simulink library "Lib_Piccolo"  (R2018b)
settings: Solver=VariableStepAuto  StartTime=0.0  StopTime=10.0  RelTol=1e-3
values from neighbouring files (symbols this model uses):
  AccelErrInt2Brakes = 0.15    [SimulationControlConfig16P.m]    (also in SimulationControlConfig16P_LEGACY.m; SimulationControlConfigTAILLESS.m = 0.2; SimulationControlConfigUTAIL.m = 0.2)
  AileronMax = 25    [SimulationControlConfig16P.m]    (also in SimulationControlConfig16P_LEGACY.m; SimulationControlConfigTAILLESS.m; SimulationControlConfigUTAIL.m)
  AileronPower = 0.00268    [SimulationControlConfig16P.m]    (also in SimulationControlConfig16P_LEGACY.m; SimulationControlConfigTAILLESS.m; SimulationControlConfigUTAIL.m)
  AileronSurfaceMax = 45    [SimulationControlConfig16P.m]    (also in SimulationControlConfig16P_LEGACY.m)
  AileronTrim = 0    [SimulationControlConfig16P.m]    (also in SimulationControlConfig16P_LEGACY.m; SimulationControlConfigTAILLESS.m; SimulationControlConfigUTAIL.m)
  Alt = 1000 + TerrainHeight    [SimulationStateConfig.m]
  AltCruise_m = testPlans(testIndx).terrainElevation * 0.3048 + 200    [SimulationControlConfig16P.m]    (also in SimulationControlConfigTAILLESS.m = 1083; SimulationControlConfigUTAIL.m = testPlans(testIndx).terrainElevation * 0.3048 + 152)
  AltitudeRate2PitchCmdIntegratorInit = 0.1    [SimulationControlPre.m]
  AltMax = 10000    [SimulationControlConfig16P.m]    (also in SimulationControlConfig16P_LEGACY.m; SimulationControlConfigTAILLESS.m; SimulationControlConfigUTAIL.m)
  AltMaxAccel = 1.25    [SimulationControlConfig16P.m]    (also in SimulationControlConfig16P_LEGACY.m = 0.9; SimulationControlConfigTAILLESS.m = 1.7; SimulationControlConfigUTAIL.m = 2)
  AltMin = 0    [SimulationControlConfig16P.m]    (also in SimulationControlConfig16P_LEGACY.m; SimulationControlConfigTAILLESS.m; SimulationControlConfigUTAIL.m)
  AltRateCmd2Pitch = 0.50    (= 0.5)    [SimulationControlConfig16P.m]    (also in SimulationControlConfig16P_LEGACY.m = 0.6; SimulationControlConfigTAILLESS.m = 0.2; SimulationControlConfigUTAIL.m = 0.3)
  AltRateError2Pitch = 0.40    (= 0.4)    [SimulationControlConfig16P.m]    (also in SimulationControlConfig16P_LEGACY.m; SimulationControlConfigTAILLESS.m = 0.55; SimulationControlConfigUTAIL.m = 0.55)
  AltRateErrorInt2Pitch = 0.50    (= 0.5)    [SimulationControlConfig16P.m]    (also in SimulationControlConfig16P_LEGACY.m = 0.45; SimulationControlConfigTAILLESS.m; SimulationControlConfigUTAIL.m = 0.75)
  AltRateLpfCutOff = 3    [SimulationControlConfig16P.m]    (also in SimulationControlConfig16P_LEGACY.m; SimulationControlConfigTAILLESS.m = 2; SimulationControlConfigUTAIL.m = 2)
  AutoNosegear2Rudder = 26    [SimulationControlConfig16P.m]    (also in SimulationControlConfig16P_LEGACY.m; SimulationControlConfigTAILLESS.m = 25.2; SimulationControlConfigUTAIL.m = 14)
  b = 5.54    [SimulationControlConfig16P.m]    (also in SimulationControlConfig16P_LEGACY.m; SimulationControlConfigTAILLESS.m = 2.37; SimulationControlConfigUTAIL.m = 2.37)
  Bank2AileronIntegratorInit = 0    [SimulationControlPre.m]
  BankMax_User = BankMax_User/180*pi    (= 0.523598775598)    [SimulationControlConfig16P.m]    (also in SimulationControlConfig16P_LEGACY.m; SimulationControlConfigTAILLESS.m = 0.610865238198; SimulationControlConfigUTAIL.m = 0.628318530718)
  baseLegFlaps = 20    [SimulationControlConfig16P.m]    (also in SimulationControlConfig16P_LEGACY.m = 0; SimulationControlConfigTAILLESS.m = 15; SimulationControlConfigUTAIL.m = 10)
  C = GeneticOpt.C    [SimulationCostFunction.m]
  c = Sw/b    (= 0.841696750903)    [SimulationControlConfig16P.m]    (also in SimulationControlConfig16P_LEGACY.m; SimulationControlConfigTAILLESS.m = 0.354008438819; SimulationControlConfigUTAIL.m = 0.354008438819)
  cell2WheelFactorMG = 5.98    [SimulationSensorConfig16P_LEGACY.m]
  cell2WheelFactorNG = 1    [SimulationSensorConfig16P_LEGACY.m]
  cellSatMaxMG = 15000    [SimulationSensorConfig16P.m]    (also in SimulationSensorConfig16P_LEGACY.m; SimulationSensorConfigTAILLESS7P.m; SimulationSensorConfigUTAIL7P.m)
  cellSatMaxNG = 1000    [SimulationSensorConfig16P.m]    (also in SimulationSensorConfig16P_LEGACY.m; SimulationSensorConfigTAILLESS7P.m; SimulationSensorConfigUTAIL7P.m)
  cellSatMinMG = -15000    [SimulationSensorConfig16P.m]    (also in SimulationSensorConfig16P_LEGACY.m; SimulationSensorConfigTAILLESS7P.m; SimulationSensorConfigUTAIL7P.m)
  cellSatMinNG = -1000    [SimulationSensorConfig16P.m]    (also in SimulationSensorConfig16P_LEGACY.m; SimulationSensorConfigTAILLESS7P.m; SimulationSensorConfigUTAIL7P.m)
  CL_Limit = CL_Max    (= 0.54)    [SimulationControlConfig16P.m]    (also in SimulationControlConfig16P_LEGACY.m; SimulationControlConfigTAILLESS.m; SimulationControlConfigUTAIL.m = 0.53)
  CL_Max = 0.54    [SimulationControlConfig16P.m]    (also in SimulationControlConfig16P_LEGACY.m; SimulationControlConfigTAILLESS.m; SimulationControlConfigUTAIL.m = 0.53)
  CL_Max_Nom = 0.465    [SimulationControlConfig16P.m]    (also in SimulationControlConfig16P_LEGACY.m; SimulationControlConfigTAILLESS.m = 0.39; SimulationControlConfigUTAIL.m)
  CL_Min = 0    [SimulationControlConfig16P.m]    (also in SimulationControlConfig16P_LEGACY.m; SimulationControlConfigTAILLESS.m; SimulationControlConfigUTAIL.m)
  ClimbMaxFraction = 0.35    [SimulationControlConfig16P.m]    (also in SimulationControlConfig16P_LEGACY.m = 0.24; SimulationControlConfigTAILLESS.m = 0.19; SimulationControlConfigUTAIL.m = 0.21)
  ClimboutMaxBank = 7.0    (= 7)    [SimulationControlConfig16P.m]    (also in SimulationControlConfig16P_LEGACY.m; SimulationControlConfigTAILLESS.m = 5; SimulationControlConfigUTAIL.m)
  ClimboutTimer = 7.0    (= 7)    [SimulationControlConfig16P.m]    (also in SimulationControlConfig16P_LEGACY.m; SimulationControlConfigTAILLESS.m; SimulationControlConfigUTAIL.m)
  dCl_per_dFlap = 0.005581818    [SimulationControlConfig16P.m]    (also in SimulationControlConfig16P_LEGACY.m = 0; SimulationControlConfigTAILLESS.m = 0; SimulationControlConfigUTAIL.m = 0)
  DecelerationCmd = 3.1    [SimulationControlConfig16P.m]    (also in SimulationControlConfig16P_LEGACY.m; SimulationControlConfigTAILLESS.m = 0.1; SimulationControlConfigUTAIL.m = 0.1)
  DeRotateLogicEndTimer = abs((NoseDownLimit_Deg-1)/DeRotateRamp_Dps)    [SimulationControlConfig16P.m]    (also in SimulationControlConfig16P_LEGACY.m; SimulationControlConfigTAILLESS.m; SimulationControlConfigUTAIL.m)
  DeRotateLogicHoldNoseUpTimer = 0.1    [SimulationControlConfig16P.m]    (also in SimulationControlConfig16P_LEGACY.m; SimulationControlConfigTAILLESS.m; SimulationControlConfigUTAIL.m)
  DeRotateLogicTimerTimeout = 2    [SimulationControlConfig16P.m]    (also in SimulationControlConfig16P_LEGACY.m; SimulationControlConfigTAILLESS.m; SimulationControlConfigUTAIL.m)
  DeRotateLowerCmdSaturation = 0    [SimulationControlConfig16P.m]    (also in SimulationControlConfig16P_LEGACY.m; SimulationControlConfigTAILLESS.m; SimulationControlConfigUTAIL.m)
  DeRotateRamp_Dps = 3    [SimulationControlConfig16P.m]    (also in SimulationControlConfig16P_LEGACY.m; SimulationControlConfigTAILLESS.m = 8; SimulationControlConfigUTAIL.m = 8)
  DeRotateUpperCmdSaturation = 7    [SimulationControlConfig16P.m]    (also in SimulationControlConfig16P_LEGACY.m; SimulationControlConfigTAILLESS.m; SimulationControlConfigUTAIL.m)
  DescentMaxFraction = 0.22    [SimulationControlConfig16P.m]    (also in SimulationControlConfig16P_LEGACY.m = 0.2; SimulationControlConfigTAILLESS.m = 0.17; SimulationControlConfigUTAIL.m = 0.17)
  DesktopSimTerrainOffset_m = 0.406    [SimulationAircraftConfig.m]
  downwindFlaps = 0    [SimulationControlConfig16P.m]    (also in SimulationControlConfig16P_LEGACY.m; SimulationControlConfigTAILLESS.m; SimulationControlConfigUTAIL.m)
  DP_init = 0.5*1.225*V_init^2    [SimulationControlConfig16P.m]    (also in SimulationControlConfig16P_LEGACY.m; SimulationControlConfigTAILLESS.m; SimulationControlConfigUTAIL.m)
  dscNoiseMG = 1    [SimulationSensorConfig16P_LEGACY.m]
  dscNoiseNG = 0.25    [SimulationSensorConfig16P_LEGACY.m]
  DSCnumBits = 24    [SimulationSensorConfig16P.m]    (also in SimulationSensorConfig16P_LEGACY.m; SimulationSensorConfigTAILLESS7P.m; SimulationSensorConfigUTAIL7P.m)
  DSCRangeMaxMG = 15000    [SimulationSensorConfig16P.m]    (also in SimulationSensorConfig16P_LEGACY.m; SimulationSensorConfigTAILLESS7P.m; SimulationSensorConfigUTAIL7P.m)
  DSCRangeMaxNG = 1000    [SimulationSensorConfig16P.m]    (also in SimulationSensorConfig16P_LEGACY.m; SimulationSensorConfigTAILLESS7P.m; SimulationSensorConfigUTAIL7P.m)
  DSCRangeMinMG = -15000    [SimulationSensorConfig16P.m]    (also in SimulationSensorConfig16P_LEGACY.m; SimulationSensorConfigTAILLESS7P.m; SimulationSensorConfigUTAIL7P.m)
  DSCRangeMinNG = -1000    [SimulationSensorConfig16P.m]    (also in SimulationSensorConfig16P_LEGACY.m; SimulationSensorConfigTAILLESS7P.m; SimulationSensorConfigUTAIL7P.m)
  dt = DLLSim.dt    [SimulationTimeStep.m]    (also in SimulationTrim.m = 0.02)
  EarlyTouchdownThreshold = 3.0    (= 3)    [SimulationControlConfig16P.m]    (also in SimulationControlConfig16P_LEGACY.m; SimulationControlConfigTAILLESS.m = 2.2; SimulationControlConfigUTAIL.m = 2.5)
  ElevatorDeflectionRate = 15    [SimulationControlConfig16P.m]    (also in SimulationControlConfig16P_LEGACY.m = 12; SimulationControlConfigTAILLESS.m = 10; SimulationControlConfigUTAIL.m = 12)
  ElevatorMax = 25    [SimulationControlConfig16P.m]    (also in SimulationControlConfig16P_LEGACY.m; SimulationControlConfigTAILLESS.m; SimulationControlConfigUTAIL.m)
  ElevatorPower = -0.002209    [SimulationControlConfig16P.m]    (also in SimulationControlConfig16P_LEGACY.m; SimulationControlConfigTAILLESS.m = -0.002956; SimulationControlConfigUTAIL.m = -0.00205983)
  ElevatorTrim = -3.5    [SimulationControlConfig16P.m]    (also in SimulationControlConfig16P_LEGACY.m; SimulationControlConfigTAILLESS.m = -6; SimulationControlConfigUTAIL.m = -8)
  elevonBias = 0    [SimulationControlConfig16P.m]    (also in SimulationControlConfig16P_LEGACY.m; SimulationControlConfigTAILLESS.m; SimulationControlConfigUTAIL.m)
  Enable_TAS_Protection = 0    [SimulationControlConfig16P.m]    (also in SimulationControlConfig16P_LEGACY.m; SimulationControlConfigTAILLESS.m; SimulationControlConfigUTAIL.m)
  EnableCrossTrackAbort = 1    [SimulationControlConfig16P.m]    (also in SimulationControlConfigTAILLESS.m; SimulationControlConfigUTAIL.m)
  EnergyBandwidth = 0.02    [SimulationControlConfig16P.m]    (also in SimulationControlConfig16P_LEGACY.m; SimulationControlConfigTAILLESS.m = 0.06; SimulationControlConfigUTAIL.m = 0.06)
  EngineLhFuelCut = 0    [SimulationAircraftConfig.m]
  EngineRhFuelCut = 0    [SimulationAircraftConfig.m]
  FastThrottleRate = 0.075    [SimulationControlConfig16P.m]    (also in SimulationControlConfig16P_LEGACY.m = 0.05; SimulationControlConfigTAILLESS.m = 0.1; SimulationControlConfigUTAIL.m = 0.1)
  FilterWarmUpTime = 2    [SimulationSensorConfig16P.m]    (also in SimulationSensorConfig16P_LEGACY.m; SimulationSensorConfigTAILLESS7P.m; SimulationSensorConfigUTAIL7P.m)
  finalApproachFlaps = 20    [SimulationControlConfig16P.m]    (also in SimulationControlConfig16P_LEGACY.m = 0; SimulationControlConfigTAILLESS.m = 22; SimulationControlConfigUTAIL.m = 10)
  FinalDescentSlope_Deg = testPlans(testIndx).descentSlope    [SimulationControlConfig16P.m]    (also in SimulationControlConfig16P_LEGACY.m; SimulationControlConfigTAILLESS.m; SimulationControlConfigUTAIL.m)
  flapMax = 0    [SimulationControlConfig16P.m]    (also in SimulationControlConfig16P_LEGACY.m; SimulationControlConfigTAILLESS.m; SimulationControlConfigUTAIL.m)
  flapRate = 7.5    [SimulationControlConfig16P.m]    (also in SimulationControlConfig16P_LEGACY.m; SimulationControlConfigTAILLESS.m = 6.6; SimulationControlConfigUTAIL.m)
  FlareHeight = 5    [SimulationControlConfig16P.m]    (also in SimulationControlConfig16P_LEGACY.m = 4.8; SimulationControlConfigTAILLESS.m = 2.5; SimulationControlConfigUTAIL.m = 2)
  FlareVerticalRate_mps = -0.4    [SimulationControlConfig16P.m]    (also in SimulationControlConfig16P_LEGACY.m = -0.5; SimulationControlConfigTAILLESS.m = -0.15; SimulationControlConfigUTAIL.m = -0.15)
  Fp_Aileron = 0.55*2*pi*RollRateLpfCutoff*dt    [SimulationControlConfig16P.m]    (also in SimulationControlConfig16P_LEGACY.m; SimulationControlConfigTAILLESS.m; SimulationControlConfigUTAIL.m)
  Fp_Alt = 0.55*AltBandwidth    (= 0.099)    [SimulationControlConfig16P.m]    (also in SimulationControlConfig16P_LEGACY.m; SimulationControlConfigTAILLESS.m = 0.587477826221; SimulationControlConfigUTAIL.m = 0.69115038379)
  Fp_AltRate = 0.55*2*pi*AltRateLpfCutOff*dt    [SimulationControlConfig16P.m]    (also in SimulationControlConfig16P_LEGACY.m; SimulationControlConfigTAILLESS.m; SimulationControlConfigUTAIL.m)
  Fp_Elevator = 0.55*2*pi*PitchRateLpfCutoff*dt    [SimulationControlConfig16P.m]    (also in SimulationControlConfig16P_LEGACY.m; SimulationControlConfigTAILLESS.m; SimulationControlConfigUTAIL.m)
  Fp_Energy = 0.55*2*pi*EnergyBandwidth    (= 0.069115038379)    [SimulationControlConfig16P.m]    (also in SimulationControlConfig16P_LEGACY.m; SimulationControlConfigTAILLESS.m = 0.207345115137; SimulationControlConfigUTAIL.m = 0.207345115137)
  Fp_Energy2 = 0.55*2*pi*EnergyBandwidth*dt    [SimulationControlConfig16P.m]    (also in SimulationControlConfig16P_LEGACY.m; SimulationControlConfigTAILLESS.m; SimulationControlConfigUTAIL.m)
  Fp_Pitch = 0.55*2*pi*PitchBandwidth    (= 2.76460153516)    [SimulationControlConfig16P.m]    (also in SimulationControlConfig16P_LEGACY.m = 3.11017672705; SimulationControlConfigTAILLESS.m = 3.80132711084; SimulationControlConfigUTAIL.m = 2.41902634326)
  Fp_Pitch_2 = 0.55*2*pi*PitchBandwidth*dt    [SimulationControlConfig16P.m]    (also in SimulationControlConfig16P_LEGACY.m; SimulationControlConfigTAILLESS.m; SimulationControlConfigUTAIL.m)
  Fp_Roll = RollBandwidth^2    (= 1)    [SimulationControlConfig16P.m]    (also in SimulationControlConfig16P_LEGACY.m = 1.44; SimulationControlConfigTAILLESS.m; SimulationControlConfigUTAIL.m)
  Fp_Rudder = 0.55*2*pi*YawRateLpfCutoff*dt    [SimulationControlConfig16P.m]    (also in SimulationControlConfig16P_LEGACY.m; SimulationControlConfigTAILLESS.m; SimulationControlConfigUTAIL.m)
  Fp_TAS = 0.55*2*pi*TASBandwidth    (= 0.103672557568)    [SimulationControlConfig16P.m]    (also in SimulationControlConfig16P_LEGACY.m; SimulationControlConfigTAILLESS.m = 0.172787595947; SimulationControlConfigUTAIL.m = 0.172787595947)
  Fp_TAS_Filter = 2*pi*TasLpfCutoff*dt    [SimulationControlConfig16P.m]    (also in SimulationControlConfig16P_LEGACY.m; SimulationControlConfigTAILLESS.m; SimulationControlConfigUTAIL.m)
  Fp_Turn = 0.55*2*pi*TurnErrLPFcutoff    (= 0.0345575191895)    [SimulationControlConfig16P.m]    (also in SimulationControlConfig16P_LEGACY.m; SimulationControlConfigTAILLESS.m = 0.172787595947; SimulationControlConfigUTAIL.m = 0.172787595947)
  Fp_TurnDerr = 0.55*2*pi*TurnDerivativeLPFcutoff    (= 0.0345575191895)    [SimulationControlConfig16P.m]    (also in SimulationControlConfig16P_LEGACY.m; SimulationControlConfigTAILLESS.m = 0.172787595947; SimulationControlConfigUTAIL.m = 0.172787595947)
  FTV = 3    [SimulationAircraftConfig.m]
  ftvStaticPositionError = 1/1.18    (= 0.847457627119)    [SimulationSensorConfig16P.m]    (also in SimulationSensorConfig16P_LEGACY.m; SimulationSensorConfigTAILLESS7P.m = 1; SimulationSensorConfigUTAIL7P.m = 1)
  g = 9.81    [SimulationStateConfig.m]
  GustSpd_Kts = testPlans(testIndx).gustSpd    [SimulationStateConfig.m]
  GustTriggerVal = testPlans(testIndx).gustTriggerVal    [SimulationStateConfig.m]
  HeadingErr2TurnRate = 0.5    [SimulationControlConfig16P.m]    (also in SimulationControlConfig16P_LEGACY.m; SimulationControlConfigTAILLESS.m; SimulationControlConfigUTAIL.m)
  HeadingErrDer2TurnRate = 0.3    [SimulationControlConfig16P.m]    (also in SimulationControlConfig16P_LEGACY.m; SimulationControlConfigTAILLESS.m; SimulationControlConfigUTAIL.m)
  IASbounce = IASstall*0.8    [SimulationControlPre.m]
  IAScruiseCMD = sqrt(2*m*9.81/(1.225*Sw*CL_cruise))    [SimulationControlConfig16P.m]    (also in SimulationControlConfig16P_LEGACY.m; SimulationControlConfigTAILLESS.m; SimulationControlConfigUTAIL.m)
  IASfinalCMD = 1.12 * IASmin    [SimulationControlConfig16P.m]    (also in SimulationControlConfig16P_LEGACY.m = 1.10 * IASmin; SimulationControlConfigTAILLESS.m = 1.10 * IASmin; SimulationControlConfigUTAIL.m = 1.15 * IASmin)
  IASflareCMD = IASstall    [SimulationControlConfig16P.m]    (also in SimulationControlConfig16P_LEGACY.m; SimulationControlConfigTAILLESS.m; SimulationControlConfigUTAIL.m)
  IASmax = 64    [SimulationControlConfig16P.m]    (also in SimulationControlConfig16P_LEGACY.m = 46; SimulationControlConfigTAILLESS.m = 38.58; SimulationControlConfigUTAIL.m = 35)
  IASmin = sqrt(2*m*9.81/(1.225*Sw*0.9*CL_Max_Nom))    [SimulationControlConfig16P.m]    (also in SimulationControlConfig16P_LEGACY.m; SimulationControlConfigTAILLESS.m; SimulationControlConfigUTAIL.m)
  IASshortCMD = IASstall    [SimulationControlConfig16P.m]    (also in SimulationControlConfig16P_LEGACY.m; SimulationControlConfigTAILLESS.m; SimulationControlConfigUTAIL.m)
  IASstall = sqrt(2*m*9.81/(1.225*Sw*CL_Max))    [SimulationControlConfig16P.m]    (also in SimulationControlConfig16P_LEGACY.m; SimulationControlConfigTAILLESS.m; SimulationControlConfigUTAIL.m)
  inFlight = 1    [SimulationControlConfig16P.m]    (also in SimulationControlConfigTAILLESS.m; SimulationControlConfigUTAIL.m)
  JetCatOffset = 5    [SimulationControlConfig16P.m]    (also in SimulationControlConfig16P_LEGACY.m)
  LaunchRollingElevator = -1.5    [SimulationControlConfig16P.m]    (also in SimulationControlConfig16P_LEGACY.m; SimulationControlConfigTAILLESS.m = 1; SimulationControlConfigUTAIL.m = 1)
  ldg_NosegearMax = 10    [SimulationControlConfig16P.m]    (also in SimulationControlConfig16P_LEGACY.m; SimulationControlConfigTAILLESS.m; SimulationControlConfigUTAIL.m)
  ldg_TrackVyErrInt2Nosegear = 0.1250    (= 0.125)    [SimulationControlConfig16P.m]    (also in SimulationControlConfig16P_LEGACY.m; SimulationControlConfigTAILLESS.m = 0.00714285714286; SimulationControlConfigUTAIL.m = 0.00714285714286)
  ldg_TrackVyErrPro2Nosegear = 0.35    [SimulationControlConfig16P.m]    (also in SimulationControlConfig16P_LEGACY.m; SimulationControlConfigTAILLESS.m = 0.0546666666667; SimulationControlConfigUTAIL.m = 0.0546666666667)
  ldg_TrackY2Vy = 0.07    [SimulationControlConfig16P.m]    (also in SimulationControlConfig16P_LEGACY.m; SimulationControlConfigTAILLESS.m = 0.17; SimulationControlConfigUTAIL.m = 0.17)
  ldg_Vy2NosegearScalingPower = 1.075    [SimulationControlConfig16P.m]    (also in SimulationControlConfig16P_LEGACY.m; SimulationControlConfigTAILLESS.m = 0.6; SimulationControlConfigUTAIL.m = 0.5)
  ldg_Y2VyScalingPower = 0.175    [SimulationControlConfig16P.m]    (also in SimulationControlConfig16P_LEGACY.m; SimulationControlConfigTAILLESS.m = 0; SimulationControlConfigUTAIL.m = 0)
  ldg_YawRate2Nosegear = 0.175    [SimulationControlConfig16P.m]    (also in SimulationControlConfig16P_LEGACY.m; SimulationControlConfigTAILLESS.m = 0.065; SimulationControlConfigUTAIL.m = 0.065)
  LiftSlope = 0.064285    [SimulationControlConfig16P.m]    (also in SimulationControlConfig16P_LEGACY.m; SimulationControlConfigTAILLESS.m = 0.058631; SimulationControlConfigUTAIL.m)
  LPFaileronInit = 0    [SimulationControlPre.m]
  LPFclestInit = 0    [SimulationControlPre.m]
  LPFenergyFFInit = 0    [SimulationControlPre.m]
  LPFtasInit = V_init + 2    [SimulationControlPre.m]
  LPFthrottleInit = ThrottleTrim    [SimulationControlPre.m]
  LPFturnErrInit = 0    [SimulationControlPre.m]
  ... (+115 more)
undefined symbols (not defined in the file or in its folder): abortFlag, alphaHPF, apmDelay, BRWNOUT, CRAWOR, CRAWUR, DiscIntNeverNeededParam, DLLSim, DLLSimStep, ECOMOR, ECOMUR, Fp_Tas, GustTrigger_HeightAgl_m, IPSTAT, LCINTEG, Ldg_Persist_Time, LOWER_FLAGS, MSG_ENABLE, NoiseStd, OLDVAL, OVERRIDE_ENABLE, OVERRIDE_VALUE, REBOOT, reversionEnable, revIASMax, revIASMin, revPitchMax, revPitchMin, revPitchRateMax, revRollMax, revRollRateMax, SAMPLE, SCALON, SensorModel, sigbuilder_block, Sim_Vx, Sim_Vy, Sim_Vz, Sim_Xpos, Sim_Ypos, Sim_Zpos, SYSOR, SYSUR, TARE, TEMPOR, TEMPUR, testIndx, testPlan, testPlans, Trim_piccoloInCmd, Trim_REFSI_FD_IN_nmodeCgShifterCmd_Ft, Trim_REFSI_FD_IN_nmodeFlapLhIBCmd_Deg, Trim_REFSI_FD_IN_nmodeFlapLhOBCmd_Deg, Trim_REFSI_FD_IN_nmodeFlapRhIBCmd_Deg, Trim_REFSI_FD_IN_nmodeFlapRhOBCmd_Deg, Trim_REFSI_FD_IN_nmodeSlatLhCmd_Deg, Trim_REFSI_FD_IN_nmodeSlatRhCmd_Deg, Trim_REFSI_FD_IN_nmodeSplrLhInbdCmd_Deg, Trim_REFSI_FD_IN_nmodeSplrLhOutbdCmd_Deg ... (+5)
libraries: simulink x866, aerolibconvert2 x60, $bdroot x52, aerolibatmos2 x5, dspswit3 x5, simulink_extras x4, dsparch4 x2, Lib_Piccolo_Alt x2, eeGeneralControl x1, dspindex x1
(part 12 of 44)

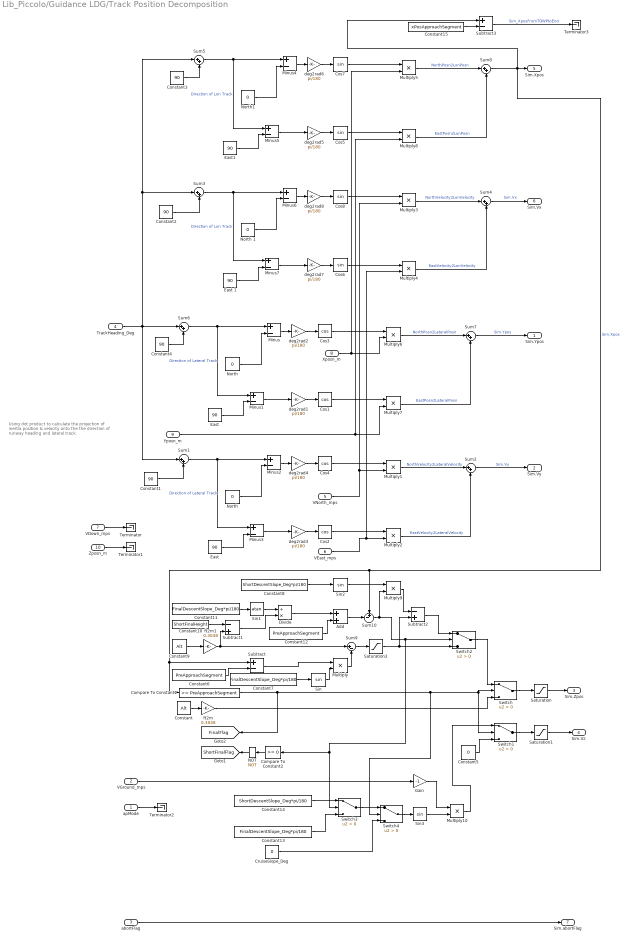
== system Lib_Piccolo/Guidance LDG/Track Position Decomposition ==
  note: Using dot product to calculate the projection of inertia position & velocity onto the
      | the direction of runway heading and lateral track
  apMode : Inport
  VGround_mps : Inport  Port=2
  abortFlag : Inport  Port=3
  TrackHeading_Deg : Inport  Port=4
  VNorth_mps : Inport  Port=5
  VEast_mps : Inport  Port=6
  VDown_mps : Inport  Port=7
  "Xposn_m " : Inport  Port=8
  Yposn_m : Inport  Port=9
  Zposn_m : Inport  Port=10
  Add : Sum
  Compare To Constant1 : simulink/Logic and Bit Operations/Compare To Constant  relop=>=  const=PreApproachSegment  OutDataTypeStr=uint8
  Compare To Constant2 : simulink/Logic and Bit Operations/Compare To Constant  relop=>=  const=0  OutDataTypeStr=uint8
  Constant : Constant  Value=Alt
  Constant{1..4} (4 alike) : Constant  Value=90
  Constant10 : Constant  Value=ShortFinalHeight
  Constant11 : Constant  Value=FinalDescentSlope_Deg*pi/180
  Constant12 : Constant  Value=PreApproachSegment
  Constant13 : Constant  Value=FinalDescentSlope_Deg*pi/180
  Constant14 : Constant  Value=ShortDescentSlope_Deg*pi/180
  Constant15 : Constant  Value=xPosApproachSegment
  Constant5 : Constant  Value=0
  Constant6 : Constant  Value=PreApproachSegment
  Constant7 : Constant  Value=FinalDescentSlope_Deg*pi/180
  Constant8 : Constant  Value=ShortDescentSlope_Deg*pi/180
  Constant9 : Constant  Value=Alt
  Cos{1..4} (4 alike) : Trigonometry  Operator=cos
  Cos{5..8} (4 alike) : Trigonometry
  CruiseSlope_Deg : Constant  Value=0
  Divide : Product  Inputs=/*
  East : Constant  Value=90
  "East " : Constant  Value=90
  East 1 : Constant  Value=90
  East1 : Constant  Value=90
  Gain : Gain  Gain=-1
  Minus{,1..7} (8 alike) : Sum  Inputs=+-
  Multiply{,1..10} (11 alike) : Product
  NOT : Logic  Operator=NOT  IconShape=distinctive  AllPortsSameDT=off  OutDataTypeStr=boolean
  North : Constant  Value=0
  "North " : Constant  Value=0
  North 1 : Constant  Value=0
  North1 : Constant  Value=0
  Saturation : Saturate  UpperLimit=AltMax  LowerLimit=TerrainHeight*0.3048
  Saturation1 : Saturate  UpperLimit=100  LowerLimit=-100
  Saturation2 : Saturate  UpperLimit=AltMax  LowerLimit=ShortFinalHeight
  Sin : Trigonometry
  Sin1 : Trigonometry  Operator=atan
  Sin2 : Trigonometry
  Sin3 : Trigonometry
  Subtract : Sum  Inputs=+-
  Subtract1 : Sum  Inputs=-+
  Subtract2 : Sum  Inputs=-+
  Subtract3 : Sum  Inputs=+-
  Sum{1..8} (8 alike) : Sum  Inputs=|++
  Sum10 : Sum  Inputs=+-|
  Sum9 : Sum  Inputs=|+-
  Switch{,1..4} (5 alike) : Switch  Criteria=u2 > Threshold
  Terminator{,1..3} (4 alike) : Terminator
  deg2rad{1..8} (8 alike) : Gain  Gain=pi/180
  ft2m : Gain  Gain=0.3048
  ft2m1 : Gain  Gain=0.3048
  Sim.Ypos : Outport
  "Sim.Vy " : Outport  Port=2
  Sim.Zpos : Outport  Port=3
  Sim.Vz : Outport  Port=4
  Sim.Xpos : Outport  Port=5
  Sim.Vx : Outport  Port=6
  Sim.abortFlag : Outport  Port=7
  tag scope: FinalFlag=global, ShortFinalFlag=global
  wires:
  Subtract3/1 -> Terminator3/1  "Sim_XposFromTDWPtoEnd"
  Constant15/1 -> Subtract3/2
  Cos1/1 -> Multiply7/1
  Yposn_m/1 -> Multiply8/2, Multiply7/2
  Multiply7/1 -> Sum7/2  "EastPosn2LateralPosn"
  Multiply6/1 -> Sum7/1  "NorthPosn2LateralPosn"
  Sum6/1 -> Minus/1, Minus1/1  "Direction of Lateral Track"
  Constant4/1 -> Sum6/2
  Cos3/1 -> Multiply6/1
  "Xposn_m "/1 -> Multiply5/2, Multiply6/2
  Sum7/1 -> Sim.Ypos/1  "Sim.Ypos"
  North/1 -> Minus/2
  Minus/1 -> deg2rad2/1
  Minus1/1 -> deg2rad1/1
  East/1 -> Minus1/2
  deg2rad2/1 -> Cos3/1
  deg2rad1/1 -> Cos1/1
  Sum2/1 -> "Sim.Vy "/1  "Sim.Vy"
  VNorth_mps/1 -> Multiply3/2, Multiply1/2
  Constant1/1 -> Sum1/2
  Cos4/1 -> Multiply1/1
  Multiply2/1 -> Sum2/2  "EastVelocity2LateralVelocity"
  Multiply1/1 -> Sum2/1  "NorthVelocity2LateralVelocity"
  VEast_mps/1 -> Multiply4/2, Multiply2/2
  Minus2/1 -> deg2rad4/1
  "North "/1 -> Minus2/2
  Minus3/1 -> deg2rad3/1
  "East "/1 -> Minus3/2
  deg2rad3/1 -> Cos2/1
  Sum1/1 -> Minus2/1, Minus3/1  "Direction of Lateral Track"
  deg2rad4/1 -> Cos4/1
  Cos2/1 -> Multiply2/1
  Constant/1 -> ft2m/1
  Zposn_m/1 -> Terminator1/1
  Minus7/1 -> deg2rad7/1
  Multiply8/1 -> Sum8/2  "EastPosn2LonPosn"
  Cos6/1 -> Multiply4/1
  deg2rad8/1 -> Cos8/1
  deg2rad7/1 -> Cos6/1
  Minus4/1 -> deg2rad6/1
  Minus5/1 -> deg2rad5/1
  Sum3/1 -> Minus6/1, Minus7/1  "Direction of Lon Track"
  TrackHeading_Deg/1 -> Sum6/1, Sum3/1, Sum5/1, Sum1/1
  North 1/1 -> Minus6/2
  Constant3/1 -> Sum5/2
  North1/1 -> Minus4/2
  East1/1 -> Minus5/2
  Constant2/1 -> Sum3/2
  Cos8/1 -> Multiply3/1
  deg2rad5/1 -> Cos5/1
  Sum5/1 -> Minus4/1, Minus5/1  "Direction of Lon Track"
  deg2rad6/1 -> Cos7/1
  Minus6/1 -> deg2rad8/1
  Multiply5/1 -> Sum8/1  "NorthPosn2LonPosn"
  Cos5/1 -> Multiply8/1
  East 1/1 -> Minus7/2
  Multiply3/1 -> Sum4/1  "NorthVelocity2LonVelocity"
  Cos7/1 -> Multiply5/1
  Multiply4/1 -> Sum4/2  "EastVelocity2LonVelocity"
  Sum8/1 -> Sum10/1, Compare To Constant1/1, Subtract/1, Sim.Xpos/1, Subtract3/1  "Sim.Xpos"
  Sum4/1 -> Sim.Vx/1  "Sim.Vx"
  Saturation/1 -> Sim.Zpos/1
  ft2m/1 -> Switch/3
  Constant5/1 -> Switch1/3
  Saturation1/1 -> Sim.Vz/1
  Switch1/1 -> Saturation1/1
  Switch/1 -> Saturation/1
  Constant6/1 -> Subtract/2
  Constant7/1 -> Sin/1
  Subtract/1 -> Multiply/1
  Sin/1 -> Multiply/2
  Constant9/1 -> ft2m1/1
  ft2m1/1 -> Subtract1/2, Sum9/1
  Multiply/1 -> Sum9/2
  Sum9/1 -> Saturation2/1
  Constant10/1 -> Subtract1/1
  Constant11/1 -> Sin1/1
  Sin1/1 -> Divide/1
  Subtract1/1 -> Divide/2
  VDown_mps/1 -> Terminator/1
  Divide/1 -> Add/1
  Constant12/1 -> Add/2
  Add/1 -> Sum10/2
  Saturation2/1 -> Subtract2/2, Switch2/3
  Constant8/1 -> Sin2/1
  Sin2/1 -> Multiply9/1
  Sum10/1 -> Switch3/2, Compare To Constant2/1, Switch2/2, Multiply9/2
  Multiply9/1 -> Subtract2/1
  Subtract2/1 -> Switch2/1
  Switch2/1 -> Switch/1
  Switch3/1 -> Switch4/1
  CruiseSlope_Deg/1 -> Switch4/3
  Switch4/1 -> Sin3/1
  VGround_mps/1 -> Gain/1
  Sin3/1 -> Multiply10/2
  Gain/1 -> Multiply10/1
  Multiply10/1 -> Switch1/1
  Constant14/1 -> Switch3/1
  Constant13/1 -> Switch3/3
  apMode/1 -> Terminator2/1
  Compare To Constant2/1 -> NOT/1
  NOT/1 -> [ShortFinalFlag]
  abortFlag/1 -> Sim.abortFlag/1
  Compare To Constant1/1 -> Switch4/2, Switch/2, Switch1/2, [FinalFlag]

== system Lib_Piccolo/Guidance Takeoff & Flight/Track Position Decomposition ==
  apMode : Inport
  VGround_mps : Inport  Port=2
  abortFlag : Inport  Port=3
  TrackHeading_Deg : Inport  Port=4
  VNorth_mps : Inport  Port=5
  VEast_mps : Inport  Port=6
  VDown_mps : Inport  Port=7
  "Xposn_m " : Inport  Port=8
  Yposn_m : Inport  Port=9
  Zposn_m : Inport  Port=10
  Flight Guidance : Subsystem
  Landing Guidance : Subsystem
  Terminator{,1..8} (9 alike) : Terminator
  Sim.Ypos : Outport
  "Sim.Vy " : Outport  Port=2
  Sim.Zpos : Outport  Port=3
  Sim.Vz : Outport  Port=4
  Sim.Xpos : Outport  Port=5
  Sim.Vx : Outport  Port=6
  Sim.abortFlag : Outport  Port=7
  wires:
  Zposn_m/1 -> Terminator1/1
  VDown_mps/1 -> Terminator/1
  apMode/1 -> Terminator2/1
  abortFlag/1 -> Sim.abortFlag/1
  TrackHeading_Deg/1 -> Landing Guidance/1(TrackHeading_Deg), Flight Guidance/1(TrackHeading_Deg)  "TrackHeading_Deg"
  "Xposn_m "/1 -> Landing Guidance/2(Xposn_m), Flight Guidance/2(Xposn_m)  "Xposn_m"
  Yposn_m/1 -> Landing Guidance/3(Yposn_m), Flight Guidance/3(Yposn_m)  "Yposn_m"
  VNorth_mps/1 -> Landing Guidance/4(VNorth_mps), Flight Guidance/4(VNorth_mps)
  VEast_mps/1 -> Landing Guidance/5(VEast_mps), Flight Guidance/5(VEast_mps)
  VGround_mps/1 -> Landing Guidance/6(VGround_mps), Flight Guidance/6(VGround_mps)  "VGround_mps"
  Flight Guidance/1(Sim.Xpos) -> Sim.Xpos/1
  Flight Guidance/2(Sim.Vx) -> Sim.Vx/1
  Flight Guidance/3(Sim.Ypos) -> Sim.Ypos/1
  Flight Guidance/4(Sim.Vy) -> "Sim.Vy "/1
  Flight Guidance/5(Sim.Zpos) -> Sim.Zpos/1
  Flight Guidance/6(Sim.Vz) -> Sim.Vz/1
  Landing Guidance/1(Sim.Xpos) -> Terminator3/1
  Landing Guidance/2(Sim.Vx) -> Terminator4/1
  Landing Guidance/3(Sim.Ypos) -> Terminator5/1
  Landing Guidance/4(Sim.Vy) -> Terminator6/1
  Landing Guidance/5(Sim.Zpos) -> Terminator7/1
  Landing Guidance/6(Sim.Vz) -> Terminator8/1

== system Lib_Piccolo/Heading Control/LPF Heading ==
  Input : Inport
  Reset : Inport  Port=2
  Add1 : Sum  Inputs=++|
  Compare To Constant2 : simulink/Logic and Bit Operations/Compare To Constant  relop=>  const=0  OutDataTypeStr=uint8
  Constant11 : Constant  Value=TurnErrLPFcutoff
  Switch1 : Switch  Criteria=u2 > Threshold
  Unit Delay1 : UnitDelay  InitialCondition=LPFturnErrInit  SampleTime=-1
  a1 : Gain  Gain=1-Fp_Turn
  b0 : Gain  Gain=Fp_Turn
  Output : Outport
  wires:
  Constant11/1 -> Compare To Constant2/1
  Compare To Constant2/1 -> Switch1/2
  Switch1/1 -> Output/1
  Input/1 -> b0/1, Switch1/3
  Add1/1 -> Switch1/1, Unit Delay1/1
  a1/1 -> Add1/1
  b0/1 -> Add1/2
  Unit Delay1/1 -> a1/1

== system Lib_Piccolo/Heading Control/LPF HeadingDerivative ==
  Input : Inport
  Reset : Inport  Port=2
  Add1 : Sum  Inputs=++|
  Compare To Constant2 : simulink/Logic and Bit Operations/Compare To Constant  relop=>  const=0  OutDataTypeStr=uint8
  Constant11 : Constant  Value=TurnDerivativeLPFcutoff
  Switch1 : Switch  Criteria=u2 > Threshold
  Unit Delay1 : UnitDelay  SampleTime=-1
  a1 : Gain  Gain=1-Fp_TurnDerr
  b0 : Gain  Gain=Fp_TurnDerr
  Output : Outport
  wires:
  Constant11/1 -> Compare To Constant2/1
  Compare To Constant2/1 -> Switch1/2
  Switch1/1 -> Output/1
  Input/1 -> b0/1, Switch1/3
  Add1/1 -> Switch1/1, Unit Delay1/1
  a1/1 -> Add1/1
  b0/1 -> Add1/2
  Unit Delay1/1 -> a1/1

== system Lib_Piccolo/Heading Control/On Ground ==
  GuidanceBankCmd : Inport
  <apMode> : Inport  Port=2
  Compare To Constant1 : simulink/Logic and Bit Operations/Compare To Constant  relop=<=  const=1  OutDataTypeStr=uint8
  Compare To Constant2 : simulink/Logic and Bit Operations/Compare To Constant  relop===  const=11  OutDataTypeStr=uint8
  GroundBankCmd : Constant  Value=0
  OR : Logic  Operator=OR  IconShape=distinctive  AllPortsSameDT=off  OutDataTypeStr=boolean
  Switch : Switch  Criteria=u2 > Threshold
  BankCmd : Outport
  wires:
  Compare To Constant2/1 -> OR/1
  <apMode>/1 -> Compare To Constant1/1, Compare To Constant2/1
  GroundBankCmd/1 -> Switch/1
  GuidanceBankCmd/1 -> Switch/3
  Switch/1 -> BankCmd/1
  OR/1 -> Switch/2
  Compare To Constant1/1 -> OR/2

== system Lib_Piccolo/Heading Control/UnwindHdg ==
  REF.yaw : Inport
  Compare To Constant3 : simulink/Logic and Bit Operations/Compare To Constant  relop=>  const=180  OutDataTypeStr=boolean
  Constant : Constant  Value=360
  Subtract : Sum  Inputs=+-
  Switch : Switch  Criteria=u2 > Threshold
  Out1 : Outport
  wires:
  REF.yaw/1 -> Subtract/1, Compare To Constant3/1, Switch/3
  Compare To Constant3/1 -> Switch/2
  Switch/1 -> Out1/1
  Constant/1 -> Subtract/2
  Subtract/1 -> Switch/1

== system Lib_Piccolo/Heading Control/UnwindHdg1 ==
  REF.yaw : Inport
  Compare To Constant3 : simulink/Logic and Bit Operations/Compare To Constant  relop=>  const=180  OutDataTypeStr=boolean
  Constant : Constant  Value=360
  Subtract : Sum  Inputs=+-
  Switch : Switch  Criteria=u2 > Threshold
  Out1 : Outport
  wires:
  REF.yaw/1 -> Subtract/1, Compare To Constant3/1, Switch/3
  Compare To Constant3/1 -> Switch/2
  Switch/1 -> Out1/1
  Constant/1 -> Subtract/2
  Subtract/1 -> Switch/1

== system Lib_Piccolo/Heading Control/WindCorrectionEstimate ==
  WindSouth : Inport
  WindWest : Inport  Port=2
  Rad2Deg : Gain  Gain=180/pi
  Sqrt : Sqrt  SaturateOnIntegerOverflow=on
  Square : Math  Operator=square  SaturateOnIntegerOverflow=on
  Square1 : Math  Operator=square  SaturateOnIntegerOverflow=on
  Subtract : Sum
  Trigonometric Function2 : Trigonometry  Operator=atan2
  WindMag : Outport
  WindDir : Outport  Port=2
  wires:
  WindSouth/1 -> Square/1, Trigonometric Function2/2
  Square/1 -> Subtract/1
  Square1/1 -> Subtract/2
  Subtract/1 -> Sqrt/1
  Sqrt/1 -> WindMag/1  "Sim.WindMagnitude"
  WindWest/1 -> Square1/1, Trigonometric Function2/1
  Trigonometric Function2/1 -> Rad2Deg/1
  Rad2Deg/1 -> WindDir/1  "Sim.WindDirection"

== system Lib_Piccolo/LDG TAS Cmd/CAS2TAS ==
  In1 : Inport
  Bus Selector2 : BusSelector  OutputSignals=airDensity_kgm
  Constant : Constant  Value=1.225
  Divide : Product  Inputs=*/
  Sqrt : Sqrt  SaturateOnIntegerOverflow=on
  Out1 : Outport
  wires:
  In1/1 -> Bus Selector2/1
  Bus Selector2/1 -> Divide/2  "<airDensity_kgm>"
  Constant/1 -> Divide/1
  Divide/1 -> Sqrt/1
  Sqrt/1 -> Out1/1

== system Lib_Piccolo/LDG TAS Cmd No Offset/CAS2TAS ==
  In1 : Inport
  Bus Selector2 : BusSelector  OutputSignals=airDensity_kgm
  Constant : Constant  Value=1.225
  Divide : Product  Inputs=*/
  Sqrt : Sqrt  SaturateOnIntegerOverflow=on
  Out1 : Outport
  wires:
  In1/1 -> Bus Selector2/1
  Bus Selector2/1 -> Divide/2  "<airDensity_kgm>"
  Constant/1 -> Divide/1
  Divide/1 -> Sqrt/1
  Sqrt/1 -> Out1/1

== system Lib_Piccolo/Piccolo State Machine/Flight State Machine ==
  <apMode> : Inport
  IAS : Inport  Port=2
  GroundSpeed : Inport  Port=3
  AND : Logic  IconShape=distinctive  AllPortsSameDT=off  OutDataTypeStr=boolean
  AND1 : Logic  IconShape=distinctive  AllPortsSameDT=off  OutDataTypeStr=boolean
  Abort Logic : Subsystem
  Compare To Constant : simulink/Logic and Bit Operations/Compare To Constant  relop===  const=0  OutDataTypeStr=boolean
  Compare To Constant1 : simulink/Logic and Bit Operations/Compare To Constant  relop===  const=3.0  OutDataTypeStr=boolean
  Compare To Constant2 : simulink/Logic and Bit Operations/Compare To Constant  relop=>=  const=ClimboutTimer  OutDataTypeStr=boolean
  Compare To Constant3 : simulink/Logic and Bit Operations/Compare To Constant  relop=>=  const=0.75*IASmin  OutDataTypeStr=boolean
  Compare To Constant4 : simulink/Logic and Bit Operations/Compare To Constant  relop=>=  const=RotationSpeed  OutDataTypeStr=boolean
  Constant : Constant  Value=2
  Constant{1,3,5..6} (4 alike) : Constant
  Constant2 : Constant  Value=3
  Constant4 : Constant  Value=4
  Constant9 : Constant  Value=11
  Latch : Subsystem
  Latch1 : Subsystem
  Latch2 : Subsystem
  Switch{,1..3} (4 alike) : Switch  Criteria=u2 > Threshold
  Switch4 : Switch  Criteria=u2 > Threshold  Threshold=0.5
  Timer : Subsystem  mask{period=3}
      mask prompts: period "Period [s]"
  Unit Delay : UnitDelay  SampleTime=-1
  Unit Delay1 : UnitDelay  SampleTime=-1
  Sim.apMode : Outport
  tag scope: RotationFlag=global, TakeoffAbortFlag=global
  wires:
  GroundSpeed/1 -> Abort Logic/2(GroundSpeed)
  <apMode>/1 -> Switch3/3
  Constant/1 -> Switch/1
  Constant1/1 -> Latch/2(Enable/!Rst)
  [RotationFlag] -> AND1/1
  Latch/1(Q_Latched) -> Switch/2
  [TouchdownDetectedFlag] -> Compare To Constant/1
  Latch2/1(Q_Latched) -> Switch1/2
  Switch/1 -> Switch1/3
  Constant2/1 -> Switch1/1
  Compare To Constant1/1 -> Timer/1(Run/!Reset)
  Switch1/1 -> Compare To Constant1/1, Switch2/3
  Timer/1(timeOut_s) -> Compare To Constant2/1
  Compare To Constant2/1 -> Latch1/1(D)
  Constant3/1 -> Latch1/2(Enable/!Rst)
  Latch1/1(Q_Latched) -> Switch2/2
  Switch2/1 -> Switch4/3
  Constant4/1 -> Switch2/1
  Compare To Constant/1 -> AND/2
  Compare To Constant3/1 -> AND/1
  AND/1 -> Latch2/1(D)
  Constant5/1 -> Latch2/2(Enable/!Rst)
  Switch3/1 -> Switch/3
  Constant6/1 -> Switch3/1
  [startTaxi] -> AND1/2, Switch3/2
  AND1/1 -> Latch/1(D)
  IAS/1 -> Unit Delay/1, Abort Logic/1(IAS), Compare To Constant3/1
  Compare To Constant4/1 -> [RotationFlag]  "RotationFlag"
  Unit Delay/1 -> Compare To Constant4/1
  Switch4/1 -> Unit Delay1/1
  [TakeoffAbortFlag] -> Switch4/2
  Constant9/1 -> Switch4/1
  Abort Logic/1(Flag_TakeoffAbort) -> [TakeoffAbortFlag]
  Unit Delay1/1 -> Sim.apMode/1

== system Lib_Piccolo/Piccolo State Machine/Landing State Machine ==
  note: Moved to Vertical Track Following Guidance in Next Block
  <apMode> : Inport
  Compare To Constant1 : simulink/Logic and Bit Operations/Compare To Constant  relop=>  const=0  OutDataTypeStr=boolean
  Compare To Constant3 : simulink/Logic and Bit Operations/Compare To Constant  relop=>  const=0  OutDataTypeStr=boolean
  Constant : Constant  Value=9
  Constant1 : Constant  Value=10
  Constant2 : Constant  Value=11
  Constant3 : Constant  Value=8
  Flare Detection : Subsystem
  FlareLatch : Subsystem
  NOT1 : Logic  Operator=NOT  IconShape=distinctive  AllPortsSameDT=off  OutDataTypeStr=boolean
  NOT2 : Logic  Operator=NOT  IconShape=distinctive  AllPortsSameDT=off  OutDataTypeStr=boolean
  ShortFinal Detection : Subsystem  Commented=on
  Switch{,1..3} (4 alike) : Switch  Criteria=u2 > Threshold
  Sim.apMode : Outport
  wires:
  Compare To Constant3/1 -> NOT2/1
  [FlareFlag] -> FlareLatch/2(FlareFlag)
  Constant3/1 -> Switch3/3
  Switch1/1 -> Switch2/1
  Switch2/1 -> Sim.apMode/1  "Sim.apMode"
  [ShortFinalFlag] -> Compare To Constant1/1
  <apMode>/1 -> Switch3/1
  Constant/1 -> Switch/3
  NOT2/1 -> Switch2/2
  [FinalFlag] -> NOT1/1
  Constant1/1 -> Switch1/3
  Switch/1 -> Switch1/1
  Switch3/1 -> Switch/1
  [Pic_AP_Mode] -> FlareLatch/1(apMode)
  [TouchdownDetectedFlag] -> Compare To Constant3/1
  FlareLatch/1(FlareLatch) -> Switch1/2
  Constant2/1 -> Switch2/3
  NOT1/1 -> Switch3/2
  Compare To Constant1/1 -> Switch/2

== system Lib_Piccolo/Piccolo State Machine FLIGHT LEGACY/Flare Detection ==
  Compare To Constant : simulink/Logic and Bit Operations/Compare To Constant  relop=>  const=0  OutDataTypeStr=boolean
  Delay : Delay  DelayLength=0.04/dt  InitialCondition=Alt*0.3048
  "FlareHeight_m " : Constant  Value=FlareHeight
  Sum : Sum  Inputs=|++
  Sum1 : Sum  Inputs=|+-
  Sum2 : Sum  Inputs=|++
  Sum4 : Sum  Inputs=|+-
  Sum5 : Sum  Inputs=|+-
  Terminator10 : Terminator
  "TerrainHeight " : Constant  Value=TerrainHeight
  VehicleRestingHeight : Constant  Value=DesktopSimTerrainOffset_m
  ft to m : Gain  Gain=0.3048
  tag scope: AltAGL_m=global, FlareFlag=global
  wires:
  Sum2/1 -> Sum1/2
  Sum1/1 -> Compare To Constant/1, [FlareFlag]
  VehicleRestingHeight/1 -> Sum2/2, Sum5/2
  ft to m/1 -> Sum4/2, Sum/1
  "TerrainHeight "/1 -> ft to m/1
  Sum5/1 -> [AltAGL_m]  "AltAGL_m"
  Sum4/1 -> Sum5/1
  Compare To Constant/1 -> Terminator10/1  "Sim.FlareFlag"
  "FlareHeight_m "/1 -> Sum/2
  [Alt_m] -> Delay/1, Sum4/1
  Delay/1 -> Sum1/1
  Sum/1 -> Sum2/1

== system Lib_Piccolo/Piccolo State Machine FLIGHT LEGACY/ShortFinal Detection ==
  Compare To Constant4 : simulink/Logic and Bit Operations/Compare To Constant  relop=>  const=0  OutDataTypeStr=boolean
  ShortFinalHeight : Constant  Value=ShortFinalHeight
  Sum3 : Sum  Inputs=|+-
  tag scope: ShortFinalFlag=global
  wires:
  Compare To Constant4/1 -> [ShortFinalFlag]  "Sim.ShortFinalFlag"
  ShortFinalHeight/1 -> Sum3/2
  [Alt_m] -> Sum3/1
  Sum3/1 -> Compare To Constant4/1

== system Lib_Piccolo/Piccolo State Machine LDG/Flare Detection ==
  Compare To Constant : simulink/Logic and Bit Operations/Compare To Constant  relop=>  const=0  OutDataTypeStr=boolean
  Delay : Delay  DelayLength=0.04/dt  InitialCondition=Alt*0.3048
  "FlareHeight_m " : Constant  Value=FlareHeight
  Sum : Sum  Inputs=|++
  Sum1 : Sum  Inputs=|+-
  Sum2 : Sum  Inputs=|++
  Sum4 : Sum  Inputs=|+-
  Sum5 : Sum  Inputs=|+-
  Terminator10 : Terminator
  "TerrainHeight " : Constant  Value=TerrainHeight
  VehicleRestingHeight : Constant  Value=DesktopSimTerrainOffset_m
  ft to m : Gain  Gain=0.3048
  tag scope: AltAGL_m=global, FlareFlag=global
  wires:
  Sum2/1 -> Sum1/2
  Sum1/1 -> Compare To Constant/1, [FlareFlag]
  VehicleRestingHeight/1 -> Sum2/2, Sum5/2
  ft to m/1 -> Sum4/2, Sum/1
  "TerrainHeight "/1 -> ft to m/1
  Sum5/1 -> [AltAGL_m]  "AltAGL_m"
  Sum4/1 -> Sum5/1
  Compare To Constant/1 -> Terminator10/1  "Sim.FlareFlag"
  "FlareHeight_m "/1 -> Sum/2
  [Alt_m] -> Delay/1, Sum4/1
  Delay/1 -> Sum1/1
  Sum/1 -> Sum2/1

== system Lib_Piccolo/Piccolo State Machine LDG/FlareLatch ==
  apMode : Inport
  FlareFlag : Inport  Port=2
  Compare To Constant1 : simulink/Logic and Bit Operations/Compare To Constant  relop=>=  const=6  OutDataTypeStr=boolean
  Compare To Constant2 : simulink/Logic and Bit Operations/Compare To Constant  relop=<  const=0  OutDataTypeStr=boolean
  Latch : Subsystem
  NOT3 : Logic  Operator=NOT  IconShape=distinctive  AllPortsSameDT=off  OutDataTypeStr=boolean
  OR : Logic  Operator=OR  IconShape=distinctive  AllPortsSameDT=off  OutDataTypeStr=boolean
  Unit Delay : UnitDelay  SampleTime=-1
  FlareLatch : Outport
  wires:
  Compare To Constant2/1 -> OR/1, Latch/1(D)
  OR/1 -> NOT3/1
  FlareFlag/1 -> Compare To Constant2/1
  Latch/1(Q_Latched) -> OR/2
  NOT3/1 -> FlareLatch/1
  apMode/1 -> Unit Delay/1
  Compare To Constant1/1 -> Latch/2(Enable/!Rst)
  Unit Delay/1 -> Compare To Constant1/1

== system Lib_Piccolo/Piccolo State Machine LDG/ShortFinal Detection ==
  Compare To Constant4 : simulink/Logic and Bit Operations/Compare To Constant  relop=>  const=0  OutDataTypeStr=boolean
  ShortFinalHeight : Constant  Value=ShortFinalHeight
  Sum3 : Sum  Inputs=|+-
  tag scope: ShortFinalFlag=global
  wires:
  Compare To Constant4/1 -> [ShortFinalFlag]  "Sim.ShortFinalFlag"
  ShortFinalHeight/1 -> Sum3/2
  [Alt_m] -> Sum3/1
  Sum3/1 -> Compare To Constant4/1

== system Lib_Piccolo/Pitch to Elevator/1st Order Reference Model ==
  PitchCmd_Body : Inport
  "Pitch_Body " : Inport  Port=2
  "Scalar " : Inport  Port=3
  "PitchRateCmd_Body " : Inport  Port=4
  "PitchRateLimit_Max " : Inport  Port=5
  " PitchRateLimit_Min " : Inport  Port=6
  apMode : Inport  Port=7
  PitchRate_Body : Inport  Port=8
  Constant : Constant  Value=PitchMaxAccel
  Constant1 : Constant  Value=0
  Constant2 : Constant  Value=100
  Fp_pitch : Gain  Gain=Fp_Pitch
  Gain1 : Gain  Gain=-1
  Gain2 : Gain  Gain=180/pi
  Gain3 : Gain  Gain=180/pi
  Gain4 : Gain  Gain=180/pi
  Manual Switch : ManualSwitch
  Multiply : Product
  NOT : Logic  Operator=NOT  IconShape=distinctive  AllPortsSameDT=off  OutDataTypeStr=boolean
  OR : Logic  Operator=OR  IconShape=distinctive  AllPortsSameDT=off  OutDataTypeStr=boolean
  OR1 : Logic  Operator=OR  IconShape=distinctive  AllPortsSameDT=off  OutDataTypeStr=boolean
  PitchRate Max Accel Limit : Subsystem
  PitchRateCMD Limit : Subsystem
  Sum : Sum  Inputs=|+-
  Sum1 : Sum  Inputs=|++
  Switch : Switch  Criteria=u2 > Threshold  Threshold=0.5
  Switch1 : Switch  Criteria=u2 > Threshold  Threshold=0.5
  Terminator1 : Terminator
  Terminator2 : Terminator
  Terminator3 : Terminator
  resetCondition : Subsystem
  resetCondition1 : $bdroot/Pitch to Elevator/1st Order Reference Model/resetCondition  SystemSampleTime=-1
  PitchRateCmd_Body : Outport
  tag scope: pitchRateLimitFlag=global
  wires:
  resetCondition1/1 -> NOT/1
  resetCondition/1(Reset) -> Switch/2
  apMode/1 -> resetCondition1/1, resetCondition/1(apMode)
  PitchRate Max Accel Limit/1(Y) -> PitchRateCmd_Body/1
  Switch/1 -> PitchRate Max Accel Limit/2(u)
  OR/1 -> [pitchRateLimitFlag]  "Sim.pitchRateLimitFlag"
  PitchRateCMD Limit/2(lowerFlag) -> OR/2
  PitchRateCMD Limit/1(upperFlag) -> OR/1
  PitchRate_Body/1 -> Switch/1
  PitchRateCMD Limit/3(y) -> Switch/3
  Gain3/1 -> Terminator3/1  "Sim.pitchRateLimit_Max"
  Gain4/1 -> Terminator2/1  "Sim.pitchRateLimit_Min"
  Gain2/1 -> Terminator1/1  "Sim.pitchRateCmd_noLimits"
  Sum1/1 -> Gain2/1, PitchRateCMD Limit/2(u)
  "PitchRateCmd_Body "/1 -> Manual Switch/1
  Constant1/1 -> Manual Switch/2
  Manual Switch/1 -> Sum1/2
  " PitchRateLimit_Min "/1 -> Gain4/1, PitchRateCMD Limit/3(lo)
  "PitchRateLimit_Max "/1 -> Gain3/1, PitchRateCMD Limit/1(up)
  Gain1/1 -> PitchRate Max Accel Limit/3(lo)
  Constant/1 -> Multiply/2
  Switch1/1 -> Gain1/1, PitchRate Max Accel Limit/1(up)
  "Scalar "/1 -> Multiply/1
  Fp_pitch/1 -> Sum1/1
  Sum/1 -> Fp_pitch/1
  "Pitch_Body "/1 -> Sum/2
  PitchCmd_Body/1 -> Sum/1
  Multiply/1 -> Switch1/1  "Sim.pitchMaxAccel"
  NOT/1 -> Switch1/2
  Constant2/1 -> Switch1/3
  PitchRate Max Accel Limit/2(upperFlag) -> OR1/1
  PitchRate Max Accel Limit/3(lowerFlag) -> OR1/2
  OR1/1 -> [pitchAccelLimitFlag]  "Sim.pitchAccelLimitFlag"

== system Lib_Piccolo/Pitch to Elevator/Cm//Alpha Estimation ==
  note: 'Stiffness' here represents the slope of a linearized Cm/Alpha curve. Multiplication against alpha estimate produces an esitmated pitch moment contribution.
  note: This calculation assumes that the Cl/alpha curve crosses (0,0) in clean configuration.
  zAccel_Body : Inport
  Q : Inport  Port=2
  Constant : Constant  Value=PitchStiffness
  Constant1 : Constant  Value=dCl_per_dFlap
  Divide : Product  Inputs=*/
  Divide1 : Product  Inputs=*/
  Gain : Gain  Gain=m/Sw
  LPF CLest : Subsystem
  Lift Slope : Constant  Value=LiftSlope
  Multiply : Product
  Multiply1 : Product
  Sum : Sum  Inputs=-+|
  STIFF : Outport
  tag scope: AoA=global
  wires:
  Divide1/1 -> LPF CLest/1(Input)  "Pic_AoA"
  Sum/1 -> Divide1/1
  Multiply1/1 -> Sum/1
  Constant1/1 -> Multiply1/1
  [flapCmd] -> Multiply1/2
  LPF CLest/1(Output) -> [AoA], Multiply/2  "Pic_AoA_Filtered"
  zAccel_Body/1 -> Gain/1
  Divide/1 -> Sum/2  "Pic_CL"
  Lift Slope/1 -> Divide1/2
  Q/1 -> Divide/2
  Gain/1 -> Divide/1
  Multiply/1 -> STIFF/1  "STIFF"
  Constant/1 -> Multiply/1

== system Lib_Piccolo/Pitch to Elevator/Dimensional Elevator Power ==
  Dynamic Pressure (Avoid Small Value) : Inport
  Average Wing Chord : Constant  Value=c
  Multiply : Product  Inputs=****/
  Unit: Per Deg : Constant  Value=ElevatorPower
  Wing Area : Constant  Value=Sw
  YInertia : Constant  Value=YInertia
  CP : Outport
  wires:
  Unit: Per Deg/1 -> Multiply/4
  Multiply/1 -> CP/1
  YInertia/1 -> Multiply/5
  Average Wing Chord/1 -> Multiply/3
  Wing Area/1 -> Multiply/2
  Dynamic Pressure (Avoid Small Value)/1 -> Multiply/1

== system Lib_Piccolo/Pitch to Elevator/DynamicPLimit ==
  note: Q saturates at ~ 100mps which in IAS is 6125Pa
  apMode : Inport
  DynamicPressure_Pa : Inport  Port=2
  Compare To Constant1 : simulink/Logic and Bit Operations/Compare To Constant  relop=>=  const=5  OutDataTypeStr=uint8
  Compare To Constant2 : simulink/Logic and Bit Operations/Compare To Constant  relop=>=  const=11  OutDataTypeStr=uint8
  Compare To Constant3 : simulink/Logic and Bit Operations/Compare To Constant  relop=>=  const=10  OutDataTypeStr=uint8
  Gain : Gain  Gain=0.5 * 1.225
  Gain1 : Gain  Gain=1.1
  Gain2 : Gain  Gain=0.8
  Gain3 : Gain  Gain=0.5 * 1.225
  Latch : Subsystem
  Qmax : Constant  Value=6125
  Saturation Dynamic : simulink/Discontinuities/Saturation Dynamic  OutMin=[]  OutMax=[]  OutDataTypeStr=Inherit: Same as second input  OutDataType=fixdt(1, 16)  OutScaling=2^-10  DoSatur=off
  Square : Math  Operator=square  SaturateOnIntegerOverflow=on
  Square1 : Math  Operator=square  SaturateOnIntegerOverflow=on
  Switch : Switch  Criteria=u2 > Threshold
  Switch1 : Switch  Criteria=u2 > Threshold
  Out1 : Outport
  tag scope: Qmin=global, Qmin_Bounce=global, Qmin_Flare=global
  wires:
  Square1/1 -> Gain3/1
  [IASmin] -> Square1/1
  Gain/1 -> Gain1/1, Gain2/1
  [IASstall] -> Square/1
  Square/1 -> Gain/1
  Latch/1(Q_Latched) -> Switch1/2
  Switch1/1 -> Saturation Dynamic/3
  Gain2/1 -> Switch1/1, [Qmin_Bounce]  "Qmin_Bounce"
  Switch/1 -> Switch1/3
  Compare To Constant2/1 -> Latch/1(D)
  Compare To Constant1/1 -> Latch/2(Enable/!Rst)
  Qmax/1 -> Saturation Dynamic/1
  Gain1/1 -> Switch/1, [Qmin_Flare]  "Qmin_Flare"
  Gain3/1 -> Switch/3, [Qmin]  "Qmin"
  Compare To Constant3/1 -> Switch/2
  apMode/1 -> Compare To Constant1/1, Compare To Constant2/1, Compare To Constant3/1
  Saturation Dynamic/1 -> Out1/1
  DynamicPressure_Pa/1 -> Saturation Dynamic/2

== system Lib_Piccolo/Pitch to Elevator/Elevator Ramp Logic ==
  Elevator In : Inport
  AP Mode : Inport  Port=2
  Elevator DeRotation Ramp : Subsystem
  Elevator Rotation Ramp : Subsystem
  Elevator Out : Outport
  wires:
  Elevator Rotation Ramp/1(Elevator Out) -> Elevator Out/1
  Elevator DeRotation Ramp/1(Elevator Out) -> Elevator Rotation Ramp/1(Elevator In)
  Elevator In/1 -> Elevator DeRotation Ramp/1(Elevator In)
  AP Mode/1 -> Elevator DeRotation Ramp/2(apMode In), Elevator Rotation Ramp/2(apMode In)
